simulink model "aero2_linearization_professor_format_R2021a"  (R2021a)
settings: Solver=ode1  StartTime=0.0  StopTime=2  FixedStep=0.002  RelTol=1e-3
model workspace (MAT data in the model file):
  Kd = 3.88928113461
  Ki = 0
  Kp = 3.78162693601
  Ts = 0.002
  U_h = timeseries
  U_h.Name = 'unnamed'
  U_h.DataInfo = tsdata.datametadata
  U_h.DataInfo.Interpolation = tsdata.interpolation
  U_h.DataInfo.Interpolation.Fhandle : function handle (value not decoded)
  U_h.DataInfo.Interpolation.Name = 'linear'
  U_h.TimeInfo = tsdata.timemetadata
  U_h.TimeInfo.Length = 30001
  U_h.TimeInfo.DuplicateTimes = 0
  U_h.TimeInfo.Time_ = [0 0.002 0.004 0.006 0.008 0.01 0.012 0.014 0.016 0.018 0.02 0.022 ... (30001 elements, 30001x1)]
  U_h.TimeInfo.Initialized = 1
  U_h.QualityInfo = tsdata.qualmetadata
  U_h.Data_ = [0 0 0 0 0 0 0 0 0 0 0 0 ... (30001 elements, 30001x1)]
  U_v = timeseries
  U_v.Name = 'unnamed'
  U_v.DataInfo = tsdata.datametadata
  U_v.DataInfo.Interpolation = tsdata.interpolation
  U_v.DataInfo.Interpolation.Fhandle : function handle (value not decoded)
  U_v.DataInfo.Interpolation.Name = 'linear'
  U_v.TimeInfo = tsdata.timemetadata
  U_v.TimeInfo.Length = 30001
  U_v.TimeInfo.DuplicateTimes = 0
  U_v.TimeInfo.Time_ = [0 0.002 0.004 0.006 0.008 0.01 0.012 0.014 0.016 0.018 0.02 0.022 ... (30001 elements, 30001x1)]
  U_v.TimeInfo.Initialized = 1
  U_v.QualityInfo = tsdata.qualmetadata
  U_v.Data_ = [0 0 0 0 0 0 0 0 0 0 0 0 ... (30001 elements, 30001x1)]
  X0 = [0; 0; 0; 0]
  ki_PI_motor = 1.84164606325
  kp_PI_motor = 0.216370391856
  kw_PI_motor = 10.85985
  meas_on = 1
  tmax = 60
Description:
  | Question 3: virtual acceleration -> inverse -> signed square roots -> ideal mechanics.
  | Step a=[0.15;-0.10] rad/s^2 at 0.2 s; x(0)=0; stop 2 s.
  | Open Acceleration (rad_s2) to compare a with actual body acceleration.
  | Ideal rotor tracking: no motor loops, voltage saturation or sensor noise. Pitch envelope +/-60 deg.
settings Model: ExtModeTrigDuration=20000  Creator=MLevis  LastModifiedBy=matiasgarcia
settings DebuggingCC: UnderspecifiedInitializationDetection=Classic  MergeDetectMultiDrivingBlocksExec=none  UnconnectedInputMsg=none  UnconnectedOutputMsg=none  UnconnectedLineMsg=none
settings ModelReferenceCC: EnableRefExpFcnMdlSchedulingChecks=off  PropagateSignalLabelsOutOfModel=off
settings RTWCC: Description=Generic Real-Time Target  GPUComputeCapability=5.0  DLArmComputeVersion=20.02.1

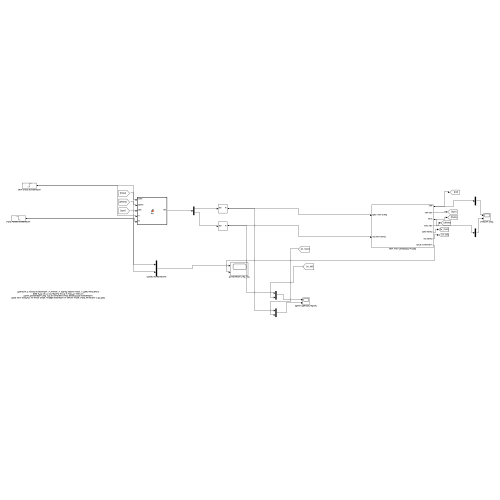
[thumbnail: Simulink's stored preview of the top-level diagram]
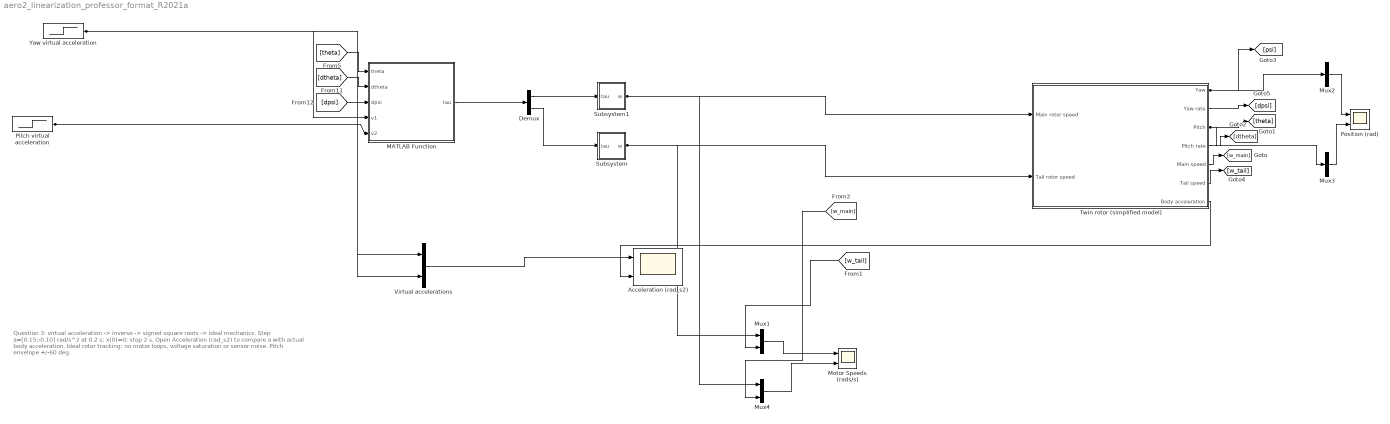
== system aero2_linearization_professor_format_R2021a ==
  note: Question 3: virtual acceleration -> inverse -> signed square roots -> ideal mechanics.
      | Step a=[0.15;-0.10] rad/s^2 at 0.2 s; x(0)=0; stop 2 s.
      | Open Acceleration (rad_s2) to compare a with actual body acceleration.
      | Ideal rotor tracking: no motor loops, voltage saturation or sensor noise. Pitch envelope +/-60 deg.
  Acceleration (rad_s2) : Scope  NumInputPorts=2
  Demux : Demux  Outputs=2
  MATLAB Function : MATLAB Function  TreatAsAtomicUnit=on
  Motor Speeds (rads/s) : Scope  NumInputPorts=2
  Mux1 : Mux  Inputs=2
  Mux2 : Mux  Inputs=1
  Mux3 : Mux  Inputs=1
  Mux4 : Mux  Inputs=2
  Pitch virtual acceleration : Step  Time=0.2  After=-0.1  SampleTime=0
  Position (rad) : Scope  NumInputPorts=2
  Subsystem : Subsystem
  Subsystem1 : Subsystem
  Twin rotor (simplified model) : Subsystem
  Virtual accelerations : Mux  Inputs=2
  Yaw virtual acceleration : Step  Time=0.2  After=0.15  SampleTime=0
  wires:
  Mux1/1 -> Motor Speeds (rads/s)/1
  Mux4/1 -> Motor Speeds (rads/s)/2
  [w_main] -> Mux4/2
  [w_tail] -> Mux1/2
  Subsystem1/1(w) -> Twin rotor (simplified model)/1(Main rotor speed), Mux4/1
  Subsystem/1(w) -> Twin rotor (simplified model)/2(Tail rotor speed), Mux1/1
  Mux2/1 -> Position (rad)/1
  Mux3/1 -> Position (rad)/2
  [theta] -> MATLAB Function/1(theta)
  [dtheta] -> MATLAB Function/2(dtheta)
  [dpsi] -> MATLAB Function/3(dpsi)
  Demux/1 -> Subsystem1/1(tau)
  Demux/2 -> Subsystem/1(tau)
  MATLAB Function/1(tau) -> Demux/1
  Twin rotor (simplified model)/1(Yaw) -> [psi], Mux2/1
  Twin rotor (simplified model)/2(Yaw rate) -> [dpsi]
  Twin rotor (simplified model)/3(Pitch) -> [theta], Mux3/1
  Twin rotor (simplified model)/4(Pitch rate) -> [dtheta]
  Twin rotor (simplified model)/5(Main speed) -> [w_main]
  Twin rotor (simplified model)/6(Tail speed) -> [w_tail]
  Yaw virtual acceleration/1 -> MATLAB Function/4(v1), Virtual accelerations/1
  Pitch virtual acceleration/1 -> MATLAB Function/5(v2), Virtual accelerations/2
  Virtual accelerations/1 -> Acceleration (rad_s2)/1
  Twin rotor (simplified model)/7(Body acceleration) -> Acceleration (rad_s2)/2

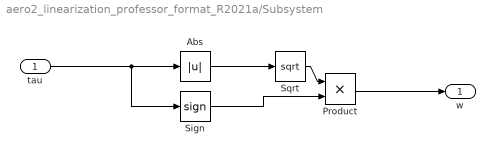
== system aero2_linearization_professor_format_R2021a/Subsystem ==
  tau : Inport
  Abs : Abs
  Product : Product
  Sign : Signum
  Sqrt : Sqrt  SaturateOnIntegerOverflow=on
  w : Outport
  wires:
  tau/1 -> Sign/1, Abs/1
  Product/1 -> w/1
  Abs/1 -> Sqrt/1
  Sqrt/1 -> Product/1
  Sign/1 -> Product/2

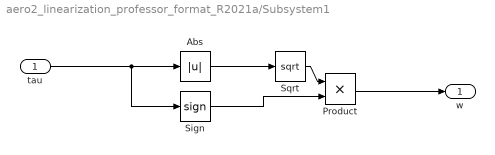
== system aero2_linearization_professor_format_R2021a/Subsystem1 ==
  tau : Inport
  Abs : Abs
  Product : Product
  Sign : Signum
  Sqrt : Sqrt  SaturateOnIntegerOverflow=on
  w : Outport
  wires:
  tau/1 -> Sign/1, Abs/1
  Product/1 -> w/1
  Abs/1 -> Sqrt/1
  Sqrt/1 -> Product/1
  Sign/1 -> Product/2

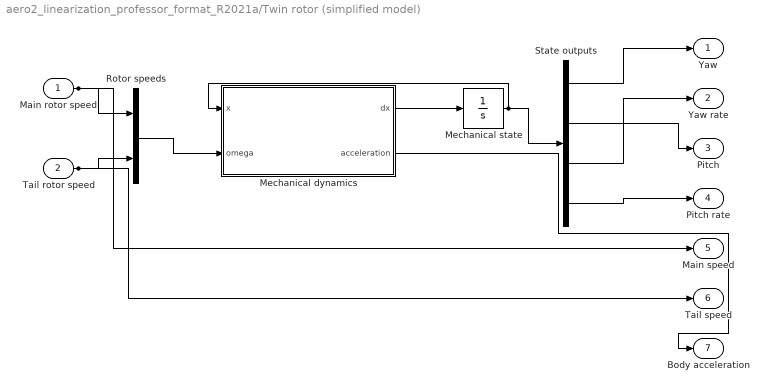
== system aero2_linearization_professor_format_R2021a/Twin rotor (simplified model) ==
  Main rotor speed : Inport
  Tail rotor speed : Inport  Port=2
  Mechanical dynamics : MATLAB Function  TreatAsAtomicUnit=on
  Mechanical state : Integrator  InitialCondition=X0
  Rotor speeds : Mux  Inputs=2
  State outputs : Demux  Outputs=[1 1 1 1]
  Yaw : Outport
  Yaw rate : Outport  Port=2
  Pitch : Outport  Port=3
  Pitch rate : Outport  Port=4
  Main speed : Outport  Port=5
  Tail speed : Outport  Port=6
  Body acceleration : Outport  Port=7
  wires:
  Main rotor speed/1 -> Rotor speeds/1, Main speed/1
  Tail rotor speed/1 -> Rotor speeds/2, Tail speed/1
  Rotor speeds/1 -> Mechanical dynamics/2(omega)
  Mechanical state/1 -> Mechanical dynamics/1(x), State outputs/1
  Mechanical dynamics/1(dx) -> Mechanical state/1
  State outputs/1 -> Yaw/1
  State outputs/3 -> Yaw rate/1
  State outputs/2 -> Pitch/1
  State outputs/4 -> Pitch rate/1
  Mechanical dynamics/2(acceleration) -> Body acceleration/1

== matlab function aero2_linearization_professor_format_R2021a/Twin rotor (simplified model)/Mechanical dynamics ==
  data: x input; dx output; omega input; acceleration output
function [dx, acceleration] = ideal_mechanics(x, omega)
fullDerivative = course_dynamics([0;0], [x;omega]);
dx = fullDerivative(1:4);
acceleration = fullDerivative(3:4);
end

function dx = course_dynamics(u, x)
%% Simplified twin-rotor model of aero2_model.pdf (2-DOF body + first-order motors)
p = struct('Jph', 0.64070000000000005, ...
    'jph', 0.01, ...
    'Jth', 0.71640000000000004, ...
    'G', 0.025399999999999999, ...
    'kT', 4.2486999999999997e-06, ...
    'kF', 2.5525999999999999e-05, ...
    'L', 0.16700000000000001, ...
    'Cor', 0.63070000000000004, ...
    'Dph', 0, ...
    'Dth', 0, ...
    'aw', 5.7800000000000002, ...
    'bw', 96.531999999999996);
dx = tr_simp_dyn(x, u, p);
end

function dx = tr_simp_dyn(x, u, p)
%TR_SIMP_DYN  Simplified twin-rotor model with voltage inputs (aero2_model.pdf).
%   Body: reduced 2-DOF model, eq. (simp)
%     Mq(th) [ddpsi; ddth] + cq + Bq dq + gq = Gamma(th) [wm|wm|; wt|wt|]
%   with cq = [-Cor sin(2th) dth dpsi; 1/2 Cor sin(2th) dpsi^2]
%   (no gyroscopic coupling, no motor reaction channel, s_m=+1, s_t=-1).
%   Rotors: first-order motor model of the hand-out
%     dw = -aw w + bw v
%   State x = [psi, theta, dpsi, dtheta, wm, wt], input u = [Um, Ut].
%   p: Jph jph Jth Dph Dth Cor L G kF kT aw bw (psim of tr_instructor_params).

    th = x(2);  dps = x(3);  dth = x(4);
    c = cos(th);  s = sin(th);
    tau = [x(5)*abs(x(5)); x(6)*abs(x(6))];

    Ms  = [p.Jph*c^2 + p.jph*s^2, 0; 0, p.Jth];
    Cs  = [-p.Cor*sin(2*th)*dth*dps; 0.5*p.Cor*sin(2*th)*dps^2];
    Ds  = [p.Dph*dps; p.Dth*dth];
    Gs  = [0; p.G*s];
    Gam = [c 0; 0 1]*[-p.kT, p.L*p.kF; p.L*p.kF, p.kT];
    ddq = Ms\(Gam*tau - Cs - Ds - Gs);

    dw  = -p.aw*x(5:6) + p.bw*u(:);
    dx  = [x(3:4); ddq; dw];
end

== matlab function aero2_linearization_professor_format_R2021a/MATLAB Function ==
  data: theta input; tau output; dtheta input; dpsi input; v1 input; v2 input
function tau = fcn(theta,dtheta,dpsi,v1,v2)
assert(abs(theta)<=pi/3,'Pitch envelope exceeded (limit 60 deg).');

Jph = 0.6407;
jph = 0.01;
Jth = 0.7164;
Dph = 0;          % B_q = 0 (aero2_model.pdf)
Dth = 0;
Cor = Jph - jph;

L = 0.167;
G = 0.0254;
kF=2.5526e-5;
kT=4.2487e-6;

M=[Jph*cos(theta)^2+jph*sin(theta)^2,0;
    0, Jth    ];
C=[-Cor*sin(2*theta)*dtheta*dpsi;
    (1/2)*Cor*sin(2*theta)*dpsi^2
  %  (1/2)*Cor*(2*theta)*dpsi^2
    ];

D=[Dph*dpsi;Dth*dtheta];

Grav=[0;
    G*sin(theta)];
Gamma=[cos(theta),0;0,1]*[-kT,L*kF;L*kF,kT];

den=L*L*kF*kF+kT*kT;
Gamma_inv=(1/den)*[-kT,L*kF;L*kF,kT]*[1/cos(theta),0;0,1];

v=[v1(1,1);v2(1,1)];

%tau=inv(Gamma)*(M*v+C+Grav);
tau=Gamma_inv*(M*v+C+D+Grav);
